simulink model "final_project"  (R2024b)
settings: Solver=FixedStepDiscrete  StartTime=0.0  StopTime=10.0  FixedStep=0.2  RelTol=1e-3
undefined symbols (not defined in the file): Kd, Ki, Kp
settings Model: Creator=Ali Saleh Al-Taher  LastModifiedBy=Ali Saleh Al-Taher

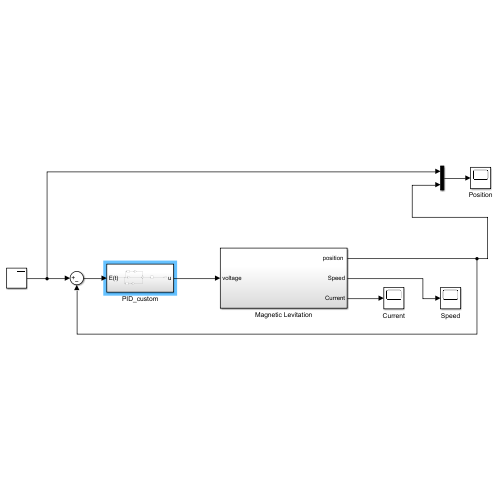
[thumbnail: Simulink's stored preview of the top-level diagram]
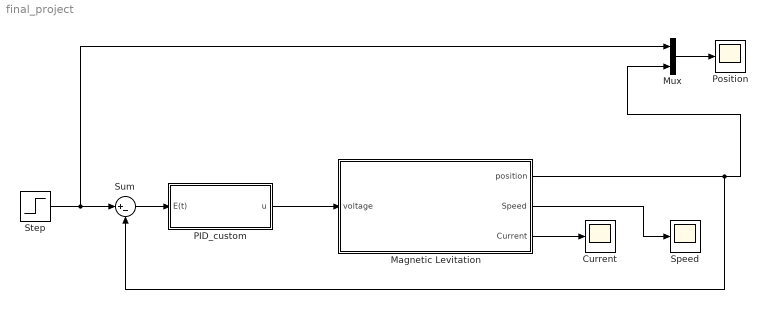
== system final_project ==
  Current : Scope
  Magnetic Levitation : Subsystem
  Mux : Mux  Inputs=2
  PID_custom : Subsystem
  Position : Scope
  Speed : Scope
  Step : Step  Time=0  After=0.06  SampleTime=0
  Sum : Sum  Inputs=|+-
  wires:
  Magnetic Levitation/3(Current) -> Current/1
  Step/1 -> Sum/1, Mux/1
  Magnetic Levitation/2(Speed) -> Speed/1
  Sum/1 -> PID_custom/1(E(t))
  PID_custom/1(u) -> Magnetic Levitation/1(voltage)
  Magnetic Levitation/1("position ") -> Mux/2, Sum/2
  Mux/1 -> Position/1

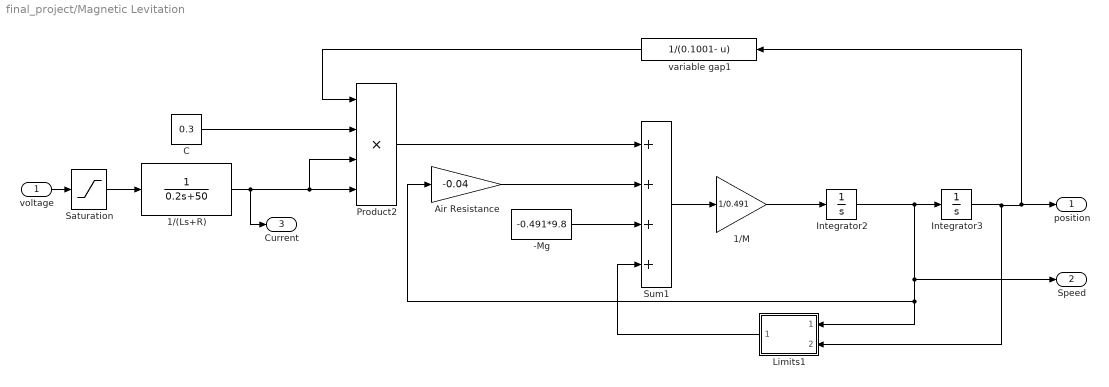
== system final_project/Magnetic Levitation ==
  voltage : Inport
  -Mg : Constant  Value=-0.491*9.8
  1/(Ls+R) : TransferFcn  Denominator=[0.2 50]
  1/M : Gain  Gain=1/0.491
  Air Resistance : Gain  Gain=-0.04
  C : Constant  Value=0.3
  Integrator2 : Integrator  LowerSaturationLimit=0
  Integrator3 : Integrator  InitialCondition=0.0001  LimitOutput=on  UpperSaturationLimit=0.1  LowerSaturationLimit=0
  Limits1 : Subsystem
      mask Display: disp('LIMIT')
  Product2 : Product  Inputs=4
  Saturation : Saturate  UpperLimit=200  LowerLimit=0  ZeroCross=off
  Sum1 : Sum  Inputs=++++
  variable gap1 : Fcn  Expr=1/(0.1001- u)
  "position " : Outport  VectorParamsAs1DForOutWhenUnconnected=off
  Speed : Outport  Port=2  VectorParamsAs1DForOutWhenUnconnected=off
  Current : Outport  Port=3  VectorParamsAs1DForOutWhenUnconnected=off
  wires:
  -Mg/1 -> Sum1/3
  1/(Ls+R)/1 -> Current/1, Product2/3, Product2/4
  Sum1/1 -> 1/M/1
  Saturation/1 -> 1/(Ls+R)/1
  Integrator2/1 -> Speed/1, Limits1/1(velocity), Air Resistance/1, Integrator3/1
  Limits1/1(force) -> Sum1/4
  C/1 -> Product2/2
  Product2/1 -> Sum1/1
  1/M/1 -> Integrator2/1
  Air Resistance/1 -> Sum1/2
  variable gap1/1 -> Product2/1
  voltage/1 -> Saturation/1
  Integrator3/1 -> Limits1/2(position), "position "/1, variable gap1/1

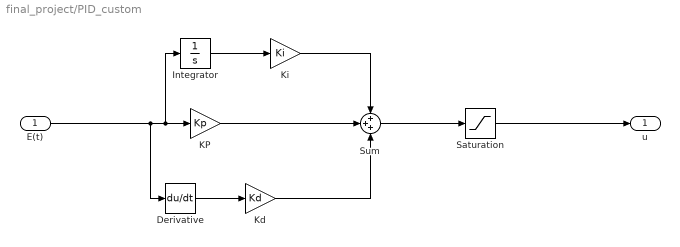
== system final_project/PID_custom ==
  E(t) : Inport
  Derivative : Derivative
  Integrator : Integrator
  KP : Gain  Gain=Kp
  Kd : Gain  Gain=Kd
  Ki : Gain  Gain=Ki
  Saturation : Saturate  UpperLimit=inf  LowerLimit=-inf
  Sum : Sum  Inputs=+++
  u : Outport
  wires:
  Integrator/1 -> Ki/1
  E(t)/1 -> Derivative/1, Integrator/1, KP/1
  Derivative/1 -> Kd/1
  KP/1 -> Sum/2
  Kd/1 -> Sum/3
  Ki/1 -> Sum/1
  Saturation/1 -> u/1
  Sum/1 -> Saturation/1

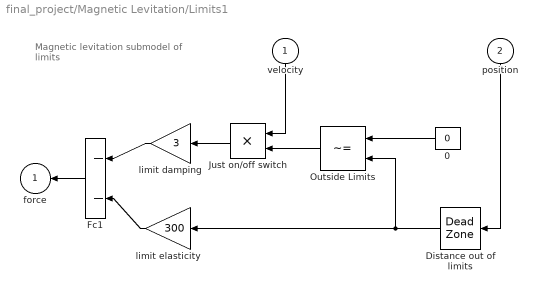
== system final_project/Magnetic Levitation/Limits1 ==
  note: Magnetic levitation
      | submodel of limits
  velocity : Inport
  position : Inport  Port=2
  0 : Constant  Value=0
  Distance out of limits : DeadZone  LowerValue=0.0002  UpperValue=0.0998  ZeroCross=off
  Fc1 : Sum  Inputs=--  InputSameDT=on  SaturateOnIntegerOverflow=on  OutDataTypeStr=Inherit: Same as first input
  "Just on/off switch " : Product  InputSameDT=on  SaturateOnIntegerOverflow=on  OutDataTypeStr=Inherit: Same as first input
  Outside Limits : RelationalOperator  Operator=~=
  limit damping : Gain  Gain=3  SaturateOnIntegerOverflow=on  OutDataTypeStr=Inherit: Same as input  ParamDataTypeStr=Inherit: Same as input
  limit elasticity : Gain  Gain=300  SaturateOnIntegerOverflow=on  OutDataTypeStr=Inherit: Same as input  ParamDataTypeStr=Inherit: Same as input
  force : Outport  VectorParamsAs1DForOutWhenUnconnected=off
  wires:
  Distance out of limits/1 -> Outside Limits/2, limit elasticity/1
  limit damping/1 -> Fc1/1
  limit elasticity/1 -> Fc1/2
  Outside Limits/1 -> "Just on/off switch "/2
  0/1 -> Outside Limits/1
  "Just on/off switch "/1 -> limit damping/1
  velocity/1 -> "Just on/off switch "/1
  Fc1/1 -> force/1
  position/1 -> Distance out of limits/1
